simulink subsystem "MotorDriveUnit_Basic_refsub"  (R2025a)
settings: Solver=VariableStepAuto  StartTime=0.0  StopTime=10.0  RelTol=1e-3
undefined symbols (not defined in the file or in its folder): Minus, motorDriveUnit, Plus
libraries: fl_lib x10, nesl_utility x7, sdl_lib x3
settings Model: Creator=isaacito  LastModifiedBy=isaacito
settings SolverCC: AlgebraicLoopSolver=TrustRegion
settings OptimizationCC: ReuseModelBlockBuffer=off
settings DebuggingCC: UnconnectedInputMsg=warning  UnconnectedOutputMsg=warning  UnconnectedLineMsg=warning
settings ModelReferenceCC: EnableRefExpFcnMdlSchedulingChecks=on
settings RTWCC: GPUComputeCapability=3.5  DLArmComputeVersion=19.05

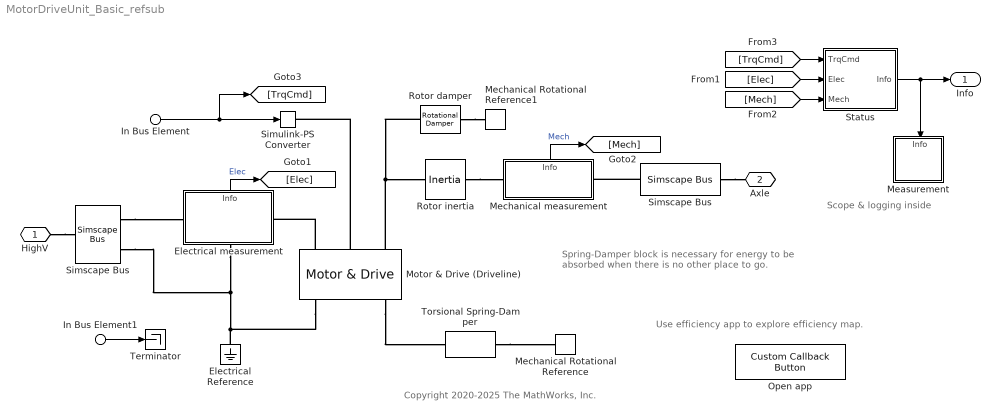
== system MotorDriveUnit_Basic_refsub ==
  note: Copyright 2020-2025 The MathWorks, Inc.
  note: Spring-Damper block is necessary
      | for energy to be absorbed when
      | there is no other place to go.
  note: Use efficiency app to explore efficiency map.
  note: Scope & logging inside
  In Bus Element : Inport  PortName=Ctrl  Element=TrqCmd
      settings: AttributesFormatString=%<Unit>
  In Bus Element1 : Inport  PortName=Ctrl  Element=HeatCmd
      settings: AttributesFormatString=%<Unit>
  " Simscape Bus" : SimscapeBus  HierarchyStrings=Plus;Minus  ConnectionType=Bus: Bus_HighVoltage
      settings: AttributesFormatString=%<ConnectionType>
  Electrical Reference : fl_lib/Electrical/Electrical Elements/Electrical Reference
  Electrical measurement : Subsystem
      settings: PortSchema="{\"entries\":[{\"content\":{\"sides\":[{\"content\":{\"connectorIds\":[\"LConn1\"]},\"type\":\"ConnectorPlacement.EquallySpacedRectSide\",\"uuid\":\"e7899a7c-736a-463f-af66-4f4d60778038\"},{\"content\":{\"connectorIds\":[\"RConn1\"],\"side\":\"RIGHT\"},\"type\":\"ConnectorPlacement.EquallySpacedRectSide\",\"uuid\":\"2a49f66b-d9e4-4ecc-9ee0-ab77c8229b93\"},{\"content\":{\"connectorIds\":[\"Out1\"],\"side\":\"TOP\"},\"type\":\"ConnectorPlacement.EquallySpacedRectSide\",\"uuid\":\"74dc25cc-80bc-4bc6-bed8-e6f8417263f8\"},{\"content\":{\"connectorIds\":[\"RConn2\"],\"side\":\"BOTTOM\"},\"type\":\"ConnectorPlacement.EquallySpacedRectSide\",\"uuid\":\"4e60d196-3559-4d10-956a-034c89d8b166\"}]},\"type\":\"ConnectorPlacement.EquallySpacedConnector\",\"uuid\":\"8c0a083e-e2f2-4f23-9344-a58537a7d46b\"}],\"packageUris\":[\"http://schema.mathworks.com/mf0/Connector/R2020b\"],\"version\":\"1.0\"}"
  Measurement : Subsystem
      settings: PortSchema="{\"entries\":[{\"content\":{\"sides\":[{\"content\":{\"connectorIds\":[]},\"type\":\"ConnectorPlacement.EquallySpacedRectSide\",\"uuid\":\"19cfde99-4be6-4a0a-8af6-ed4f14eb0886\"},{\"content\":{\"connectorIds\":[],\"side\":\"RIGHT\"},\"type\":\"ConnectorPlacement.EquallySpacedRectSide\",\"uuid\":\"3cf153af-2962-4120-ab50-e67b4416993f\"},{\"content\":{\"connectorIds\":[\"In1\"],\"side\":\"TOP\"},\"type\":\"ConnectorPlacement.EquallySpacedRectSide\",\"uuid\":\"52c8c20a-9afb-4db3-a700-9e2c1af5819c\"}]},\"type\":\"ConnectorPlacement.EquallySpacedConnector\",\"uuid\":\"028a2713-aaab-4082-ae82-0b7a26be3a8b\"}],\"packageUris\":[\"http://schema.mathworks.com/mf0/Connector/R2020b\"],\"version\":\"1.0\"}"
  Mechanical Rotational Reference : fl_lib/Mechanical/Rotational Elements/Mechanical Rotational Reference
  Mechanical Rotational Reference1 : fl_lib/Mechanical/Rotational Elements/Mechanical Rotational Reference
  Mechanical measurement : Subsystem
      settings: PortSchema="{\"entries\":[{\"content\":{\"sides\":[{\"content\":{\"connectorIds\":[\"LConn1\"]},\"type\":\"ConnectorPlacement.EquallySpacedRectSide\",\"uuid\":\"5fa31342-f07e-4673-a9a7-985a7d429b77\"},{\"content\":{\"connectorIds\":[\"RConn1\"],\"side\":\"RIGHT\"},\"type\":\"ConnectorPlacement.EquallySpacedRectSide\",\"uuid\":\"9acd2d80-16ac-46ed-87fd-cbe927805b31\"},{\"content\":{\"connectorIds\":[\"Out1\"],\"side\":\"TOP\"},\"type\":\"ConnectorPlacement.EquallySpacedRectSide\",\"uuid\":\"4cbbe886-3c02-40e0-8c42-e8f0172dc845\"},{\"content\":{\"connectorIds\":[],\"side\":\"HIDDEN\"},\"type\":\"ConnectorPlacement.EquallySpacedRectSide\",\"uuid\":\"587bbe77-2244-497b-b5ee-9581dc02e6d6\"}]},\"type\":\"ConnectorPlacement.EquallySpacedConnector\",\"uuid\":\"7667f692-53dd-486a-a403-194e7923bdd7\"}],\"packageUris\":[\"http://schema.mathworks.com/mf0/Connector/R2020b\"],\"version\":\"1.0\"}"
  Motor & Drive (Driveline) : sdl_lib/Engines & Motors/Motor & Drive  torque_max=motorDriveUnit.trqMax_Nm N*m  power_max=motorDriveUnit.powerMax_kW kW  Tc=motorDriveUnit.responseTime_s s  eff=motorDriveUnit.efficiency_pct  w_eff=motorDriveUnit.spd_eff_rpm rpm  T_eff=motorDriveUnit.trq_eff_Nm N*m  thermal_port=simscape.enum.thermaleffects.omit  thermal_mass=motorDriveUnit.thermalMass_J_perK J/K  temperature_specify=on  temperature_priority=High  temperature=initial.MDU_Temperature_K K  temperature_nominal_specify=off  temperature_nominal_value=1  temperature_nominal_unit=K
      settings: InternalSimscapePortConfiguration="{\"Bottom\":[],\"Left\":[{\"id\":\"Vp\",\"label\":\"+\",\"type\":\"foundation.electrical.electrical\"},{\"id\":\"Tr\",\"label\":\"Tr\",\"type\":\"input\"},{\"id\":\"R\",\"label\":\"R\",\"type\":\"foundation.mechanical.rotational.rotational\"}],\"Right\":[{\"id\":\"Vm\",\"label\":\"-\",\"type\":\"foundation.electrical.electrical\"},{\"id\":\"Omega\",\"label\":\"w\",\"type\":\"output\"},{\"id\":\"C\",\"label\":\"C\",\"type\":\"foundation.mechanical.rotational.rotational\"}],\"Top\":[]}"
  Open app : CustomCallbackButton  Configuration="{\"components\":[{\"name\":\"BackgroundImageComponent\",\"settings\":{\"image\":{\"size\":[0,0],\"src\":\"default\",\"srcOrientation\":\"Right\"},\"position\":[0,0,1,1]}},{\"name\":\"ButtonStateComponent\",\"settings\":{\"buttonType\":\"momentary\",\"clickFcn\":\"MotorDriveUnitEfficiencyApp_Basic\",\"onValue\":1,\"position\":[0,0,1,1],\"pressDelay\":\"500\",\"pressFcn\":\"\",\"repeatInterval\":\"0\",\"states\":[{\"horizontalAlignment\":\"center\",\"image\":{\"position\":[0,0,1,1],\"size\":[1,1],\"src\":\"default\",\"srcOrientation\":\"Right\"},\"label\":{\"color\":[0.01176470588,0.01176470588,0.01176470588,1],\"icon\":{\"size\":[0,0],\"src\":\"default\",\"srcOrientation\":\"Right\"},\"iconOffset\":0,\"iconPlacement\":\"left\",\"opacity\":1,\"show\":true,\"text\":{\"content\":\"Open app\",\"font\":\"Helvetica\"}},\"labelOffset\":[0,0],\"verticalAlignment\":\"middle\"},{\"horizontalAlignment\":\"center\",\"image\":{\"position\":[0,0,1,1],\"size\":[1,1],\"src\":\"default\",\"srcOrientation\":\"Right\"},\"label\":{\"color\":[0.01176470588,0.01176470588,0.01176470588,1],\"icon\":{\"size\":[0,0],\"src\":\"default\",\"srcOrientation\":\"Right\"},\"iconOffset\":0,\"iconPlacement\":\"left\",\"opacity\":1,\"show\":true,\"text\":{\"content\":\"Open app\",\"font\":\"Helvetica\"}},\"labelOffset\":[0,0],\"verticalAlignment\":\"middle\"},{\"horizontalAlignment\":\"center\",\"image\":{\"position\":[0,0,1,1],\"size\":[1,1],\"src\":\"default\",\"srcOrientation\":\"Right\"},\"label\":{\"color\":[0.01176470588,0.01176470588,0.01176470588,1],\"icon\":{\"size\":[0,0],\"src\":\"default\",\"srcOrientation\":\"Right\"},\"iconOffset\":0,\"iconPlacement\":\"left\",\"opacity\":1,\"show\":true,\"text\":{\"content\":\"Open app\",\"font\":\"Helvetica\"}},\"labelOffset\":[0,0],\"verticalAlignment\":\"middle\"},{\"horizontalAlignment\":\"center\",\"image\":{\"position\":[0,0,1,1],\"size\":[1,1],\"src\":\"default\",\"srcOrientation\":\"Right\"},\"label\":{\"color\":[0.01176470588,0.01176470588,0.01176470588,1],\"icon\":{\"size\":[0,0],\"src\":\"default\",\"srcOrientation\":\"Right\"},\"iconOffset\":0,\"iconPlacement\":\"left\",\"opacity\":1,\"show\":true,\"text\":{\"content\":\"Open app\",\"font\":\"Helvetica\"}},\"labelOffset\":[0,0],\"verticalAlignment\":\"middle\"}]}},{\"name\":\"ForegroundImageComponent\",\"settings\":{\"image\":{\"size\":[0,0],\"src\":\"default\",\"srcOrientation\":\"Right\"},\"isForeground\":1,\"position\":[0,0,1,1]}}],\"derived\":{\"blockParameters\":{\"AutoActivate\":true,\"ButtonText\":\"Open app\",\"ButtonType\":\"Momentary\",\"ClickFcn\":\"MotorDriveUnitEfficiencyApp_Basic\",\"OnValue\":1,\"PressDelay\":\"500\",\"PressFcn\":\"\",\"RepeatInterval\":\"0\",\"fixedAspectRatio\":\"off\"}},\"settings\":{\"BindingType\":\"standalone\",\"autoActivate\":true,\"backgroundColor\":[244,244,244,1],\"backgroundOffset\":0.2,\"backgroundOpacity\":1,\"fixedAspectRatio\":\"off\",\"foregroundColor\":[0.01176470588,0.01176470588,0.01176470588,1],\"migratedFromLegacy\":true,\"useBackgroundColor\":true,\"variant\":\"callback\",\"version\":\"R2025a\"},\"type\":\"Button\"}"  CustomBackgroundColor="{\"color\":[0.9568627450980393,0.9568627450980393,0.9568627450980393],\"show\":true}"
  Rotor damper : sdl_lib/Couplings & Drives/Springs & Dampers/Rotational Damper  D=motorDriveUnit.rotorDamping_Nm_per_radps N*m*s/rad  thermal_port=simscape.enum.thermaleffects.omit  thermal_mass=50 kJ/K  temperature_specify=off  temperature_priority=High  temperature=300 K  temperature_nominal_specify=off  temperature_nominal_value=1  temperature_nominal_unit=K
  Rotor inertia : fl_lib/Mechanical/Rotational Elements/Inertia  inertia=motorDriveUnit.rotorInertia_kg_m2 kg*m^2  num_ports=foundation.enum.numPorts2.two  w_specify=on  w_priority=High  w=initial.motorDriveUnit_RotorSpd_rpm rpm  w_nominal_specify=off  w_nominal_value=1  w_nominal_unit=rad/s  t_specify=off  t_priority=None  t=0 N*m  t_nominal_specify=off  t_nominal_value=1  t_nominal_unit=N*m
      settings: InternalSimscapePortConfiguration="{\"Bottom\":[],\"Left\":[{\"id\":\"I\",\"label\":\"\",\"type\":\"foundation.mechanical.rotational.rotational\"}],\"Right\":[{\"id\":\"J\",\"label\":\"\",\"type\":\"foundation.mechanical.rotational.rotational\"}],\"Top\":[]}"
  Simscape Bus : SimscapeBus  HierarchyStrings=AngSpd  ConnectionType=Bus: Bus_Rotational
      settings: AttributesFormatString=%<ConnectionType>
  Simulink-PS Converter : nesl_utility/Simulink-PS Converter  PhysicalDomain=network_engine_domain  SubClassName=ps_input  LeftPortType=input  RightPortType=output  PseudoPeriodic=off  Frequencies=[]  NoiseDistribution=none  NoiseParameters=[]  Unit=N*m  AffineConversion=off  FilteringAndDerivatives=filter  SimscapeFilterOrder=1  InputFilterTimeConstant=.001  UdotUserProvided=1
  Status : Subsystem
  Terminator : Terminator
  Torsional Spring-Damper : sdl_lib/Couplings & Drives/Torsional Spring-Damper  k=1000 N*m/rad  mu_visc=10000 m*N/rpm  trq_coulomb=0 N*m  static_kinetic_ratio=1.1  w_tol=0.1 rpm  model_hardstop=0  upper_bound=10 deg  lower_bound=-10 deg  hardstop_model=1  k_endstop=1e6 N*m/rad  D_endstop=10 N*m/(rad/s)  transition=0.001 rad  coeff_rest=0.7  w_tol_hardstop=0.1 rad/s  trq_tol=0.001 N*m  x0=0 deg
      settings: InternalSimscapePortConfiguration="{\"Bottom\":[],\"Left\":[{\"id\":\"R\",\"label\":\"R\",\"type\":\"foundation.mechanical.rotational.rotational\"}],\"Right\":[{\"id\":\"C\",\"label\":\"C\",\"type\":\"foundation.mechanical.rotational.rotational\"}],\"Top\":[]}"
  HighV : PMIOPort  Side=Left
  Axle : PMIOPort  Port=2  Side=Right
  Info : Outport
  wires:
  Electrical measurement/1(Info) -> [Elec]  "Elec"
  [TrqCmd] -> Status/1(TrqCmd)
  [Elec] -> Status/2(Elec)
  Mechanical measurement/1(Info) -> [Mech]  "Mech"
  In Bus Element1/1 -> Terminator/1
  [Mech] -> Status/3(Mech)
  In Bus Element/1 -> [TrqCmd], Simulink-PS Converter/1
  Status/1(Info) -> Measurement/1(Info), Info/1
  connections:
  Electrical measurement/RConn2 -- Motor & Drive (Driveline)/RConn1 -- Electrical Reference/LConn1 -- " Simscape Bus"/LConn2
  Motor & Drive (Driveline)/LConn3 -- Rotor damper/LConn1 -- Rotor inertia/RConn1
  Motor & Drive (Driveline)/LConn1 -- Electrical measurement/RConn1
  Simscape Bus/LConn1 -- Mechanical measurement/RConn1
  Motor & Drive (Driveline)/LConn2 -- Simulink-PS Converter/RConn1
  " Simscape Bus"/LConn1 -- Electrical measurement/LConn1
  HighV/RConn1 -- " Simscape Bus"/RConn1
  Torsional Spring-Damper/RConn1 -- Mechanical Rotational Reference/LConn1
  Simscape Bus/RConn1 -- Axle/RConn1
  Motor & Drive (Driveline)/RConn3 -- Torsional Spring-Damper/LConn1
  Rotor inertia/LConn1 -- Mechanical measurement/LConn1
  Rotor damper/RConn1 -- Mechanical Rotational Reference1/LConn1

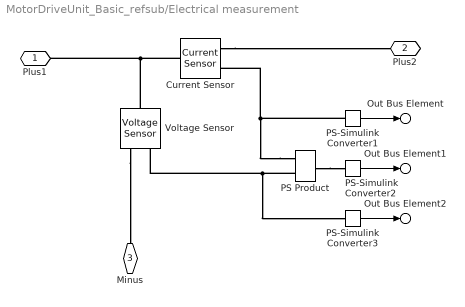
== system MotorDriveUnit_Basic_refsub/Electrical measurement ==
  Current Sensor : fl_lib/Electrical/Electrical Sensors/Current Sensor
  PS Product : fl_lib/Physical Signals/Functions/PS Product
  PS-Simulink Converter1 : nesl_utility/PS-Simulink Converter  PhysicalDomain=network_engine_domain  SubClassName=ps_output  LeftPortType=input  RightPortType=output  PseudoPeriodic=off  Frequencies=[]  VectorFormat=1-D array  Unit=A  AffineConversion=off
  PS-Simulink Converter2 : nesl_utility/PS-Simulink Converter  PhysicalDomain=network_engine_domain  SubClassName=ps_output  LeftPortType=input  RightPortType=output  PseudoPeriodic=off  Frequencies=[]  VectorFormat=1-D array  Unit=kW  AffineConversion=off
  PS-Simulink Converter3 : nesl_utility/PS-Simulink Converter  PhysicalDomain=network_engine_domain  SubClassName=ps_output  LeftPortType=input  RightPortType=output  PseudoPeriodic=off  Frequencies=[]  VectorFormat=1-D array  Unit=V  AffineConversion=off
  Voltage Sensor : fl_lib/Electrical/Electrical Sensors/Voltage Sensor
  Plus1 : PMIOPort  Side=Left
  Plus2 : PMIOPort  Port=2  Side=Right
  Minus : PMIOPort  Port=3  Side=Right
  Out Bus Element : Outport  PortName=Info  Element=Current
  Out Bus Element1 : Outport  PortName=Info  Element=ElecPower
  Out Bus Element2 : Outport  PortName=Info  Element=Voltage
  wires:
  PS-Simulink Converter1/1 -> Out Bus Element/1
  PS-Simulink Converter3/1 -> Out Bus Element2/1
  PS-Simulink Converter2/1 -> Out Bus Element1/1
  connections:
  PS Product/RConn1 -- PS-Simulink Converter2/LConn1
  PS Product/LConn1 -- Current Sensor/RConn1 -- PS-Simulink Converter1/LConn1
  Voltage Sensor/RConn1 -- PS-Simulink Converter3/LConn1 -- PS Product/LConn2
  Voltage Sensor/LConn1 -- Plus1/RConn1 -- Current Sensor/LConn1
  Current Sensor/RConn2 -- Plus2/RConn1
  Voltage Sensor/RConn2 -- Minus/RConn1

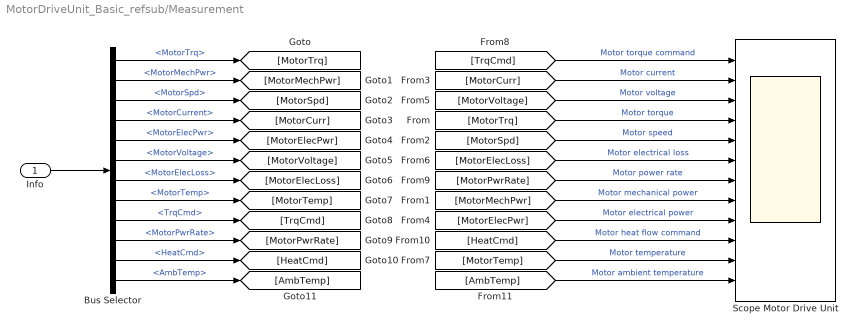
== system MotorDriveUnit_Basic_refsub/Measurement ==
  Info : Inport
  Bus Selector : BusSelector  OutputSignals=MotorTrq,MotorMechPwr,MotorSpd,MotorCurrent,MotorElecPwr,MotorVoltage,MotorElecLoss,MotorTemp,TrqCmd,MotorPwrRate,HeatCmd,AmbTemp
  Scope Motor Drive Unit : Scope  NumInputPorts=12
  wires:
  Info/1 -> Bus Selector/1
  Bus Selector/1 -> [MotorTrq]  "<MotorTrq>"
  Bus Selector/2 -> [MotorMechPwr]  "<MotorMechPwr>"
  Bus Selector/3 -> [MotorSpd]  "<MotorSpd>"
  Bus Selector/4 -> [MotorCurr]  "<MotorCurrent>"
  Bus Selector/5 -> [MotorElecPwr]  "<MotorElecPwr>"
  Bus Selector/6 -> [MotorVoltage]  "<MotorVoltage>"
  Bus Selector/7 -> [MotorElecLoss]  "<MotorElecLoss>"
  Bus Selector/8 -> [MotorTemp]  "<MotorTemp>"
  Bus Selector/9 -> [TrqCmd]  "<TrqCmd>"
  Bus Selector/10 -> [MotorPwrRate]  "<MotorPwrRate>"
  Bus Selector/11 -> [HeatCmd]  "<HeatCmd>"
  Bus Selector/12 -> [AmbTemp]  "<AmbTemp>"
  [TrqCmd] -> Scope Motor Drive Unit/1  "Motor torque command"
  [MotorCurr] -> Scope Motor Drive Unit/2  "Motor current"
  [MotorVoltage] -> Scope Motor Drive Unit/3  "Motor voltage"
  [MotorTrq] -> Scope Motor Drive Unit/4  "Motor torque"
  [MotorSpd] -> Scope Motor Drive Unit/5  "Motor speed"
  [MotorElecLoss] -> Scope Motor Drive Unit/6  "Motor electrical loss"
  [MotorPwrRate] -> Scope Motor Drive Unit/7  "Motor power rate"
  [MotorMechPwr] -> Scope Motor Drive Unit/8  "Motor mechanical power"
  [MotorElecPwr] -> Scope Motor Drive Unit/9  "Motor electrical power"
  [HeatCmd] -> Scope Motor Drive Unit/10  "Motor heat flow command"
  [MotorTemp] -> Scope Motor Drive Unit/11  "Motor temperature"
  [AmbTemp] -> Scope Motor Drive Unit/12  "Motor ambient temperature"

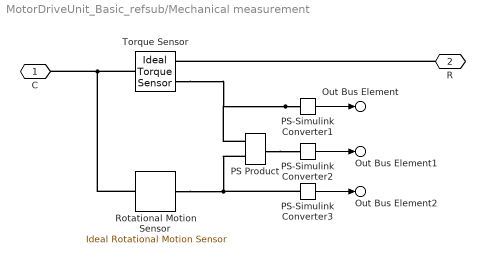
== system MotorDriveUnit_Basic_refsub/Mechanical measurement ==
  PS Product : fl_lib/Physical Signals/Functions/PS Product
  PS-Simulink Converter1 : nesl_utility/PS-Simulink Converter  PhysicalDomain=network_engine_domain  SubClassName=ps_output  LeftPortType=input  RightPortType=output  PseudoPeriodic=off  Frequencies=[]  VectorFormat=1-D array  Unit=N*m  AffineConversion=off
  PS-Simulink Converter2 : nesl_utility/PS-Simulink Converter  PhysicalDomain=network_engine_domain  SubClassName=ps_output  LeftPortType=input  RightPortType=output  PseudoPeriodic=off  Frequencies=[]  VectorFormat=1-D array  Unit=kW  AffineConversion=off
  PS-Simulink Converter3 : nesl_utility/PS-Simulink Converter  PhysicalDomain=network_engine_domain  SubClassName=ps_output  LeftPortType=input  RightPortType=output  PseudoPeriodic=off  Frequencies=[]  VectorFormat=1-D array  Unit=rpm  AffineConversion=off
  Rotational Motion Sensor : fl_lib/Mechanical/Mechanical Sensors/Ideal Rotational Motion Sensor  reference=foundation.enum.MeasurementReference.absolute  acceleration_port=false  velocity_port=true  position_port=false  wrap_angle=simscape.enum.onoff.off  offset=0 rad
      settings: InternalSimscapePortConfiguration="{\"Bottom\":[],\"Left\":[{\"id\":\"R\",\"label\":\"R\",\"type\":\"foundation.mechanical.rotational.rotational\"}],\"Right\":[{\"id\":\"W\",\"label\":\"W\",\"type\":\"output\"}],\"Top\":[]}"
  Torque Sensor : fl_lib/Mechanical/Mechanical Sensors/Ideal Torque Sensor
  C : PMIOPort  Side=Left
  R : PMIOPort  Port=2  Side=Right
  Out Bus Element : Outport  PortName=Info  Element=Trq
  Out Bus Element1 : Outport  PortName=Info  Element=MechPower
  Out Bus Element2 : Outport  PortName=Info  Element=Spd
  wires:
  PS-Simulink Converter1/1 -> Out Bus Element/1
  PS-Simulink Converter2/1 -> Out Bus Element1/1
  PS-Simulink Converter3/1 -> Out Bus Element2/1
  connections:
  PS Product/RConn1 -- PS-Simulink Converter2/LConn1
  PS-Simulink Converter3/LConn1 -- Rotational Motion Sensor/RConn1 -- PS Product/LConn2
  Torque Sensor/LConn1 -- Rotational Motion Sensor/LConn1 -- C/RConn1
  R/RConn1 -- Torque Sensor/RConn1
  PS-Simulink Converter1/LConn1 -- Torque Sensor/RConn2 -- PS Product/LConn1

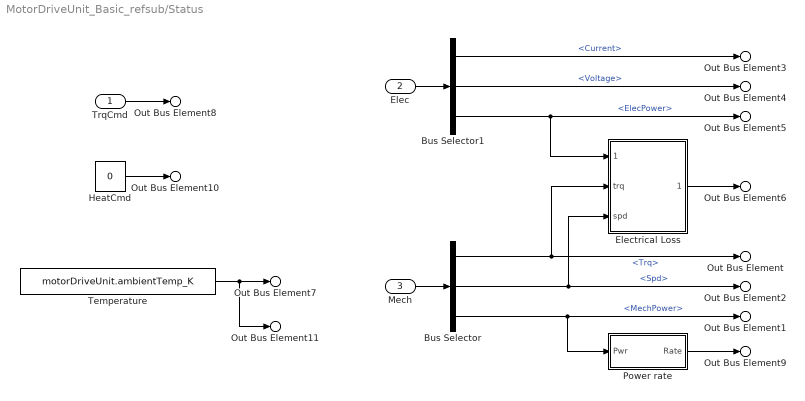
== system MotorDriveUnit_Basic_refsub/Status ==
  TrqCmd : Inport
  Elec : Inport  Port=2
  Mech : Inport  Port=3
  Bus Selector : BusSelector  OutputSignals=Trq,Spd,MechPower
  Bus Selector1 : BusSelector  OutputSignals=Current,Voltage,ElecPower
  Electrical Loss : Subsystem
  HeatCmd : Constant  Value=0
  Power rate : Subsystem
  Temperature : Constant  Value=motorDriveUnit.ambientTemp_K
  Out Bus Element : Outport  PortName=Info  Element=MotorTrq
  Out Bus Element1 : Outport  PortName=Info  Element=MotorMechPwr
  Out Bus Element2 : Outport  PortName=Info  Element=MotorSpd
  Out Bus Element3 : Outport  PortName=Info  Element=MotorCurrent
  Out Bus Element4 : Outport  PortName=Info  Element=MotorElecPwr
  Out Bus Element5 : Outport  PortName=Info  Element=MotorVoltage
  Out Bus Element6 : Outport  PortName=Info  Element=MotorElecLoss
  Out Bus Element7 : Outport  PortName=Info  Element=MotorTemp
      settings: AttributesFormatString=%<Unit>
  Out Bus Element8 : Outport  PortName=Info  Element=TrqCmd
  Out Bus Element9 : Outport  PortName=Info  Element=MotorPwrRate
  Out Bus Element10 : Outport  PortName=Info  Element=HeatCmd
  Out Bus Element11 : Outport  PortName=Info  Element=AmbTemp
      settings: AttributesFormatString=%<Unit>
  wires:
  Power rate/1(Rate) -> Out Bus Element9/1
  Electrical Loss/1(elec_loss) -> Out Bus Element6/1
  Bus Selector1/3 -> Electrical Loss/1(elec_pwr), Out Bus Element5/1  "<ElecPower>"
  Bus Selector1/2 -> Out Bus Element4/1  "<Voltage>"
  Bus Selector1/1 -> Out Bus Element3/1  "<Current>"
  Bus Selector/3 -> Power rate/1(Pwr), Out Bus Element1/1  "<MechPower>"
  Bus Selector/2 -> Electrical Loss/3(spd), Out Bus Element2/1  "<Spd>"
  Bus Selector/1 -> Out Bus Element/1, Electrical Loss/2(trq)  "<Trq>"
  TrqCmd/1 -> Out Bus Element8/1
  HeatCmd/1 -> Out Bus Element10/1
  Temperature/1 -> Out Bus Element11/1, Out Bus Element7/1
  Elec/1 -> Bus Selector1/1
  Mech/1 -> Bus Selector/1

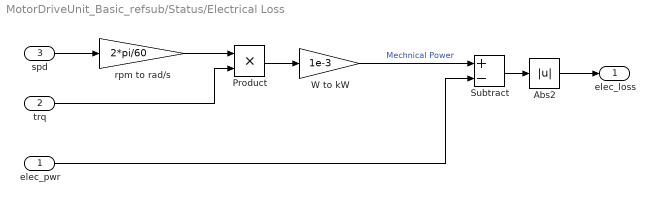
== system MotorDriveUnit_Basic_refsub/Status/Electrical Loss ==
  elec_pwr : Inport  Unit=kW
      settings: AttributesFormatString=%<Unit>
  trq : Inport  Port=2  Unit=N*m
      settings: AttributesFormatString=%<Unit>
  spd : Inport  Port=3  Unit=rpm
      settings: AttributesFormatString=%<Unit>
  Abs2 : Abs  ZeroCross=off  SaturateOnIntegerOverflow=off
  Product : Product
  Subtract : Sum  Inputs=+-
  W to kW : Gain  Gain=1e-3
  rpm to rad/s : Gain  Gain=2*pi/60
  elec_loss : Outport  Unit=kW
      settings: AttributesFormatString=%<Unit>
  wires:
  W to kW/1 -> Subtract/1  "Mechnical Power"
  Abs2/1 -> elec_loss/1
  Subtract/1 -> Abs2/1
  elec_pwr/1 -> Subtract/2
  Product/1 -> W to kW/1
  rpm to rad/s/1 -> Product/1
  spd/1 -> rpm to rad/s/1
  trq/1 -> Product/2

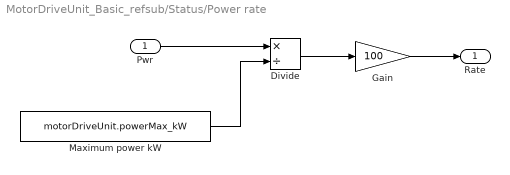
== system MotorDriveUnit_Basic_refsub/Status/Power rate ==
  Pwr : Inport  Unit=kW
      settings: AttributesFormatString=%<Unit>
  Divide : Product  Inputs=*/
  Gain : Gain  Gain=100
  Maximum power kW : Constant  Value=motorDriveUnit.powerMax_kW
  Rate : Outport  Unit=%
  wires:
  Maximum power kW/1 -> Divide/2
  Gain/1 -> Rate/1
  Divide/1 -> Gain/1
  Pwr/1 -> Divide/1
